simulink model "XAUTO02_reference"  (R2025a)
settings: Solver=FixedStepDiscrete  StartTime=0  StopTime=10  FixedStep=0.002  RelTol=1e-3
undefined symbols (not defined in the file): drive_loss_fraction, drive_loss_time, initial_speed, left_right_phase, road_amplitude, road_wavelength, speed_reference, vehicle_mass
settings Model: Creator=SimuVerity Contributors  LastModifiedBy=SimuVerity Contributors

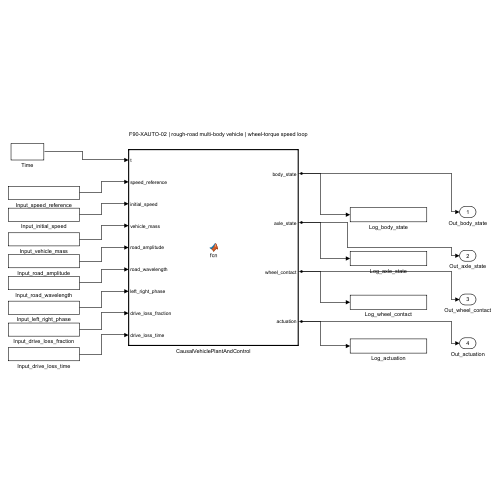
[thumbnail: Simulink's stored preview of the top-level diagram]
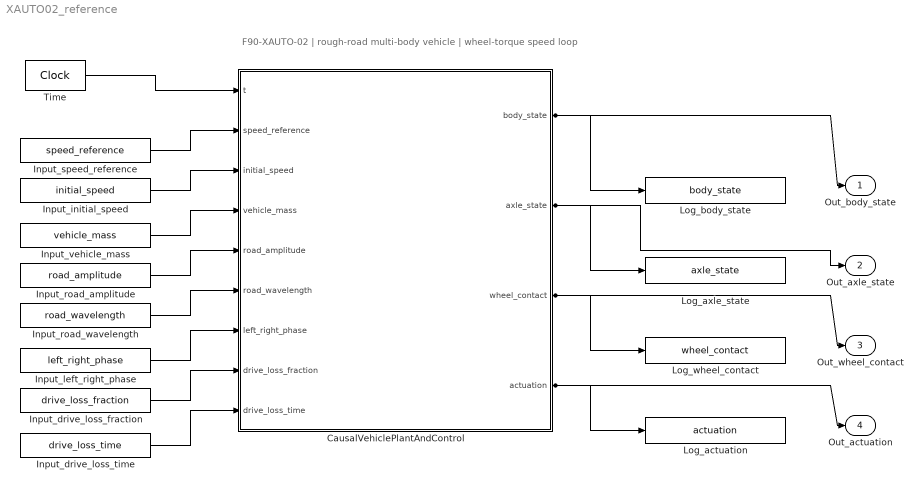
== system XAUTO02_reference ==
  note: F90-XAUTO-02 | rough-road multi-body vehicle | wheel-torque speed loop
  CausalVehiclePlantAndControl : MATLAB Function  TreatAsAtomicUnit=on
  Input_drive_loss_fraction : Constant  Value=drive_loss_fraction
  Input_drive_loss_time : Constant  Value=drive_loss_time
  Input_initial_speed : Constant  Value=initial_speed
  Input_left_right_phase : Constant  Value=left_right_phase
  Input_road_amplitude : Constant  Value=road_amplitude
  Input_road_wavelength : Constant  Value=road_wavelength
  Input_speed_reference : Constant  Value=speed_reference
  Input_vehicle_mass : Constant  Value=vehicle_mass
  Log_actuation : ToWorkspace  VariableName=actuation  SaveFormat=Timeseries  SampleTime=-1
  Log_axle_state : ToWorkspace  VariableName=axle_state  SaveFormat=Timeseries  SampleTime=-1
  Log_body_state : ToWorkspace  VariableName=body_state  SaveFormat=Timeseries  SampleTime=-1
  Log_wheel_contact : ToWorkspace  VariableName=wheel_contact  SaveFormat=Timeseries  SampleTime=-1
  Time : DigitalClock  SampleTime=0.002
  Out_body_state : Outport
  Out_axle_state : Outport  Port=2
  Out_wheel_contact : Outport  Port=3
  Out_actuation : Outport  Port=4
  wires:
  Time/1 -> CausalVehiclePlantAndControl/1(t)
  Input_speed_reference/1 -> CausalVehiclePlantAndControl/2(speed_reference)
  Input_initial_speed/1 -> CausalVehiclePlantAndControl/3(initial_speed)
  Input_vehicle_mass/1 -> CausalVehiclePlantAndControl/4(vehicle_mass)
  Input_road_amplitude/1 -> CausalVehiclePlantAndControl/5(road_amplitude)
  Input_road_wavelength/1 -> CausalVehiclePlantAndControl/6(road_wavelength)
  Input_left_right_phase/1 -> CausalVehiclePlantAndControl/7(left_right_phase)
  Input_drive_loss_fraction/1 -> CausalVehiclePlantAndControl/8(drive_loss_fraction)
  Input_drive_loss_time/1 -> CausalVehiclePlantAndControl/9(drive_loss_time)
  CausalVehiclePlantAndControl/1(body_state) -> Log_body_state/1, Out_body_state/1
  CausalVehiclePlantAndControl/2(axle_state) -> Log_axle_state/1, Out_axle_state/1
  CausalVehiclePlantAndControl/3(wheel_contact) -> Log_wheel_contact/1, Out_wheel_contact/1
  CausalVehiclePlantAndControl/4(actuation) -> Log_actuation/1, Out_actuation/1

== matlab function XAUTO02_reference/CausalVehiclePlantAndControl ==
  data: t input; body_state output; speed_reference input; initial_speed input; vehicle_mass input; road_amplitude input; road_wavelength input; left_right_phase input; drive_loss_fraction input; drive_loss_time input; axle_state output; wheel_contact output; actuation output
function [body_state,axle_state,wheel_contact,actuation] = fcn(t,speed_reference,initial_speed,vehicle_mass,road_amplitude,road_wavelength,left_right_phase,drive_loss_fraction,drive_loss_time)
%#codegen
persistent x vx zb vzb pitch pitchRate roll rollRate zf vzf rollf rollRateF zr vzr rollr rollRateR omega integ tau
dt=0.002; g=9.81; Rw=0.34; track=1.60; wheelbase=3.00;
if isempty(x) || t<0.5*dt
  x=0; vx=initial_speed; zb=0; vzb=0; pitch=0; pitchRate=0; roll=0; rollRate=0;
  zf=0; vzf=0; rollf=0; rollRateF=0; zr=0; vzr=0; rollr=0; rollRateR=0;
  omega=(initial_speed/Rw)*ones(1,4); integ=0; tau=zeros(1,4);
end
m=max(vehicle_mass,1000); ms=.78*m; mf=.11*m; mr=.11*m;
Ixx=.375*m; Iyy=1.875*m; Ixf=.050*m; Ixr=.050*m;
af=wheelbase/2; ar=wheelbase/2; halfTrack=track/2;
[hFL,hdFL]=road(x+af-12,road_amplitude,road_wavelength,0,vx);
[hFR,hdFR]=road(x+af-12,road_amplitude,road_wavelength,left_right_phase,vx);
[hRL,hdRL]=road(x-ar-12,road_amplitude,road_wavelength,0,vx);
[hRR,hdRR]=road(x-ar-12,road_amplitude,road_wavelength,left_right_phase,vx);
h=[hFL hFR hRL hRR]; hd=[hdFL hdFR hdRL hdRR];
bodyZ=[zb+af*pitch+halfTrack*roll,zb+af*pitch-halfTrack*roll,zb-ar*pitch+halfTrack*roll,zb-ar*pitch-halfTrack*roll];
bodyV=[vzb+af*pitchRate+halfTrack*rollRate,vzb+af*pitchRate-halfTrack*rollRate,vzb-ar*pitchRate+halfTrack*rollRate,vzb-ar*pitchRate-halfTrack*rollRate];
axleZ=[zf+halfTrack*rollf,zf-halfTrack*rollf,zr+halfTrack*rollr,zr-halfTrack*rollr];
axleV=[vzf+halfTrack*rollRateF,vzf-halfTrack*rollRateF,vzr+halfTrack*rollRateR,vzr-halfTrack*rollRateR];
ks=[22000 22000 27000 27000]; cs=[1800 1800 1800 1800];
Fs=ks.*(axleZ-bodyZ)+cs.*(axleV-bodyV);
kt=65000; ct=400; fz0=.25*m*g;
tireDef=h-axleZ; tireDyn=kt*tireDef+ct*(hd-axleV);
Fz=min(max(fz0+tireDyn,0),3.2*fz0); tireDyn=Fz-fz0;
slip=(Rw*omega-vx)./max(max(abs(Rw*omega),abs(vx)),0.7);
mu=.90; Fx=mu*Fz.*tanh(slip/.10);
speedError=speed_reference-vx; integ=min(max(integ+dt*speedError,-10),10);
drag=.42*vx*abs(vx); base=320*speedError+85*integ+drag*Rw/4;
targetSlip=.065*tanh(base/280); raw=base+1250*(targetSlip-slip);
lossActive=double(t>=drive_loss_time && t<drive_loss_time+1.20);
eff=max(1-drive_loss_fraction*lossActive,.20);
cmd=min(max(raw,-1150),1150);
delivered=cmd; delivered([2 4])=eff*cmd([2 4]);
tau=tau+dt*(delivered-tau)/.045;
Jw=1.95; domega=(tau-Rw*Fx-.018*omega)/Jw;
ax=(sum(Fx)-drag)/m;
azb=sum(Fs)/ms;
pitchAcc=(af*(Fs(1)+Fs(2))-ar*(Fs(3)+Fs(4)))/Iyy;
rollAcc=halfTrack*(Fs(1)-Fs(2)+Fs(3)-Fs(4))/Ixx;
azf=(tireDyn(1)+tireDyn(2)-Fs(1)-Fs(2))/mf;
azr=(tireDyn(3)+tireDyn(4)-Fs(3)-Fs(4))/mr;
rollAccF=halfTrack*((tireDyn(1)-Fs(1))-(tireDyn(2)-Fs(2)))/Ixf;
rollAccR=halfTrack*((tireDyn(3)-Fs(3))-(tireDyn(4)-Fs(4)))/Ixr;
vx=max(vx+dt*ax,0); x=x+dt*vx;
vzb=vzb+dt*azb; zb=zb+dt*vzb;
pitchRate=pitchRate+dt*pitchAcc; pitch=pitch+dt*pitchRate;
rollRate=rollRate+dt*rollAcc; roll=roll+dt*rollRate;
vzf=vzf+dt*azf; zf=zf+dt*vzf; rollRateF=rollRateF+dt*rollAccF; rollf=rollf+dt*rollRateF;
vzr=vzr+dt*azr; zr=zr+dt*vzr; rollRateR=rollRateR+dt*rollAccR; rollr=rollr+dt*rollRateR;
omega=max(omega+dt*domega,0);
slip=(Rw*omega-vx)./max(max(abs(Rw*omega),abs(vx)),0.7);
body_state=[x,vx,zb,vzb,pitch,pitchRate,roll,rollRate,ax,azb];
axle_state=[zf,vzf,rollf,rollRateF,zr,vzr,rollr,rollRateR];
wheel_contact=[omega,slip,Fz,Fx,h,tireDef];
actuation=[cmd,tau,speedError,lossActive];
end
function [height,rate]=road(s,amp,wavelength,phase,speed)
if s<=0
  height=0; rate=0;
else
  k=2*pi/max(wavelength,.5);
  ramp=min(s/6,1); dramp=double(s<6)/6;
  carrier=.68*sin(k*s+phase)+.32*sin(1.73*k*s+.4*phase);
  dcarrier=.68*k*cos(k*s+phase)+.32*1.73*k*cos(1.73*k*s+.4*phase);
  height=amp*ramp*carrier; rate=amp*(dramp*carrier+ramp*dcarrier)*speed;
end
end
